simulink model "pcssp_KCURR_RZIp_MUSCLE3"  (R2025b)
settings: Solver=VariableStepAuto  StartTime=t_start  StopTime=t_max  RelTol=1e-3
values from neighbouring files (symbols this model uses):
  CSPF_volt_cmd_FF = (coils_resistance(cspf_coil_idx) .* reference_current(1,cspf_coil_idx))'    [muscle_controller_NICE_IMAS_iter_init.m]
  enable_KCURR = 1    [muscle_controller_NICE_IMAS_iter_init.m]
  enable_RZIp = 1    [muscle_controller_NICE_IMAS_iter_init.m]
  IpControlMode_KCURR = 1    [muscle_controller_NICE_IMAS_iter_init.m]
  IpControlMode_RZIp = 0    [muscle_controller_NICE_IMAS_iter_init.m]
  schedulingVar_KCURR = 0    [muscle_controller_NICE_IMAS_iter_init.m]
  schedulingVar_RZIp = [50, 1, 1.2]'    [muscle_controller_NICE_IMAS_iter_init.m]
Description:
  | The KCURR_PFPO1 module implements a CS/PF current controller, including control of IpThis version performs internal gain scheduling based on an externally fed scheduling variable. Note: the coils are sorted as CS3U CS2U CS1 CS2L CS3L P1 P2 P3 P4 P5 P6
settings Model: DataDictionary=pcssp_KCURR_PFPO1.sldd  Creator=ravenst1  LastModifiedBy=sanderm
settings DebuggingCC: UnderspecifiedInitializationDetection=Classic  MergeDetectMultiDrivingBlocksExec=none
settings ModelReferenceCC: PropagateSignalLabelsOutOfModel=off

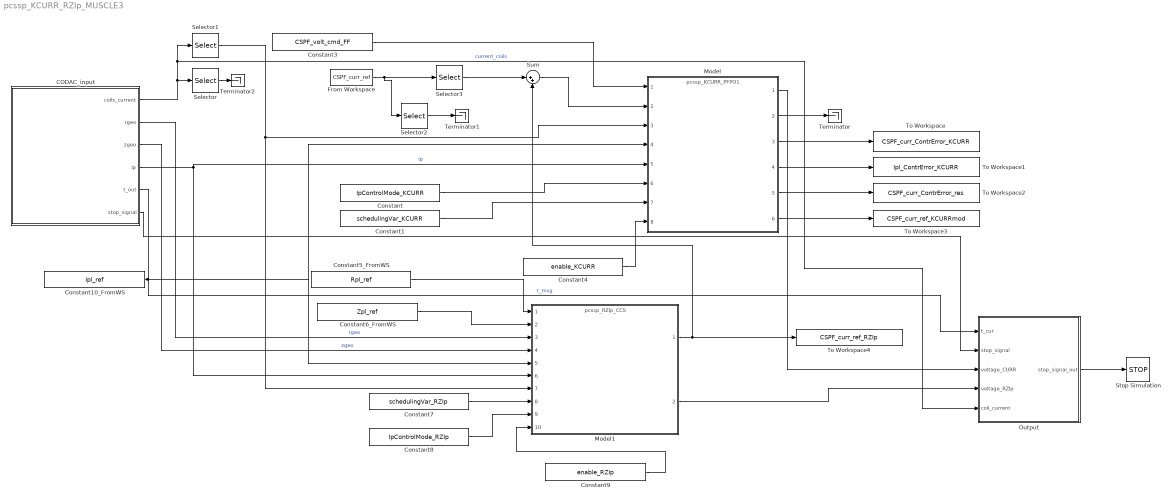
== system pcssp_KCURR_RZIp_MUSCLE3 ==
  CODAC_input : MATLAB Function  TreatAsAtomicUnit=on
  Constant : Constant  Value=IpControlMode_KCURR  OutDataTypeStr=boolean
  Constant1 : Constant  Value=schedulingVar_KCURR
  Constant10_FromWS : FromWorkspace  VariableName=Ipl_ref
  Constant3 : Constant  Value=CSPF_volt_cmd_FF
  Constant4 : Constant  Value=enable_KCURR
  Constant5_FromWS : FromWorkspace  VariableName=Rpl_ref
  Constant6_FromWS : FromWorkspace  VariableName=Zpl_ref
  Constant7 : Constant  Value=schedulingVar_RZIp
  Constant8 : Constant  Value=IpControlMode_RZIp  OutDataTypeStr=boolean
  Constant9 : Constant  Value=enable_RZIp  OutDataTypeStr=boolean
  From Workspace : FromWorkspace  VariableName=CSPF_curr_ref
  Model : ModelReference  ModelNameDialog=pcssp_KCURR_PFPO1.slx  SimulationMode=Normal  ModelReferenceVersion=6.1
  Model1 : ModelReference  ModelNameDialog=pcssp_RZIp_CCS.slx  SimulationMode=Normal  ModelReferenceVersion=1.1
  Output : MATLAB Function  TreatAsAtomicUnit=on
  Selector : Selector  IndexMode=Zero-based  InputPortWidth=14  IndexOptions=Index vector (dialog)  Indices=[12 13]  OutputSizes=1
  Selector1 : Selector  IndexMode=Zero-based  InputPortWidth=14  IndexOptions=Index vector (dialog)  Indices=[0 1 2 4 5 6 7 8 9 10 11]  OutputSizes=1
  Selector2 : Selector  IndexMode=Zero-based  InputPortWidth=14  IndexOptions=Index vector (dialog)  Indices=[12 13]  OutputSizes=1
  Selector3 : Selector  IndexMode=Zero-based  InputPortWidth=14  IndexOptions=Index vector (dialog)  Indices=[0 1 2 4 5 6 7 8 9 10 11]  OutputSizes=1
  Stop Simulation : Stop
  Sum : Sum  Inputs=|++
  Terminator : Terminator
  Terminator1 : Terminator
  Terminator2 : Terminator
  To Workspace : ToWorkspace  VariableName=CSPF_curr_ContrError_KCURR  SaveFormat=Timeseries  SampleTime=-1
  To Workspace1 : ToWorkspace  VariableName=Ipl_ContrError_KCURR  SaveFormat=Timeseries  SampleTime=-1
  To Workspace2 : ToWorkspace  VariableName=CSPF_curr_ContrError_res  SaveFormat=Timeseries  SampleTime=-1
  To Workspace3 : ToWorkspace  VariableName=CSPF_curr_ref_KCURRmod  SaveFormat=Timeseries  SampleTime=-1
  To Workspace4 : ToWorkspace  VariableName=CSPF_curr_ref_RZIp  SaveFormat=Timeseries  SampleTime=-1
  wires:
  CODAC_input/1(coils_current) -> Output/5(coil_current), Selector1/1, Selector/1  "current_coils"
  Model/1 -> Output/3(voltage_CURR)
  Constant3/1 -> Model/1
  Model/3 -> To Workspace/1
  Model/4 -> To Workspace1/1
  Model/5 -> To Workspace2/1
  Model/6 -> To Workspace3/1
  Constant4/1 -> Model/8
  Constant1/1 -> Model/7
  Constant/1 -> Model/6
  CODAC_input/2(rgeo) -> Model1/3  "rgeo"
  CODAC_input/3(zgeo) -> Model1/4  "zgeo"
  CODAC_input/4(ip) -> Model1/6, Model/5  "ip"
  Constant9/1 -> Model1/10
  Constant8/1 -> Model1/9
  Constant7/1 -> Model1/8
  Model1/2 -> Output/4(voltage_RZIp)
  From Workspace/1 -> Selector2/1, Selector3/1
  Selector2/1 -> Terminator1/1
  Selector/1 -> Terminator2/1
  Selector1/1 -> Model1/7, Model/3
  CODAC_input/5(t_out) -> Output/1(t_cur)  "t_msg"
  CODAC_input/6(stop_signal) -> Output/2(stop_signal)
  Model/2 -> Terminator/1
  Model1/1 -> To Workspace4/1, Sum/2
  Selector3/1 -> Sum/1
  Sum/1 -> Model/2
  Output/1(stop_signal_out) -> Stop Simulation/1
  Constant10_FromWS/1 -> Model1/5, Model/4
  Constant5_FromWS/1 -> Model1/1
  Constant6_FromWS/1 -> Model1/2

== matlab function pcssp_KCURR_RZIp_MUSCLE3/Output ==
  data: t_cur input; stop_signal input; voltage_CURR input; voltage_RZIp input; stop_signal_out output; coil_current input
function stop_signal_out = CODAC_output(t_cur, stop_signal, voltage_CURR,voltage_RZIp,coil_current)

% initialize to prevent simulink errors
% pellet_trigger = 0;

voltage=voltage_CURR+voltage_RZIp;

% constrain python function to run extrinsically in Matlab (no codegen)
coder.extrinsic('muscle_NICE_input');

muscle_NICE_input(t_cur,voltage,coil_current);

stop_signal_out = stop_signal;

== matlab function pcssp_KCURR_RZIp_MUSCLE3/CODAC_input ==
  data: coils_current output; rgeo output; zgeo output; ip output; t_out output; stop_signal output
function [coils_current,rgeo,zgeo, ip, t_out, stop_signal] = CODAC_input

% initialize to prevent simulink errors
coils_current=zeros(14,1);
rgeo = 0;
zgeo = 0;
ip= 0;
t_out = 0;
stop_signal = 0;

% constrain python function to run extrinsically in Matlab (no codegen)
coder.extrinsic('muscle_IDS_NICE_output');

% receive the data
[coils_current,rgeo,zgeo,ip,t_out,stop_signal] = muscle_IDS_NICE_output();

%coils_current=coils_current';

end
